simulink model "A_Identification_CSTR_open"  (R2024b)
settings: Solver=ode15s  StartTime=0.0  StopTime=100  RelTol=1e-3
settings Model: Creator=User  LastModifiedBy=HP
settings SolverCC: AlgebraicLoopSolver=TrustRegion
settings DebuggingCC: UnconnectedInputMsg=warning  UnconnectedOutputMsg=warning  UnconnectedLineMsg=warning
settings ModelReferenceCC: EnableRefExpFcnMdlSchedulingChecks=on
settings SFSimCC: CustomCodeUndefinedFunction=UseInterfaceOnly
settings RTWCC: GPUComputeCapability=3.5

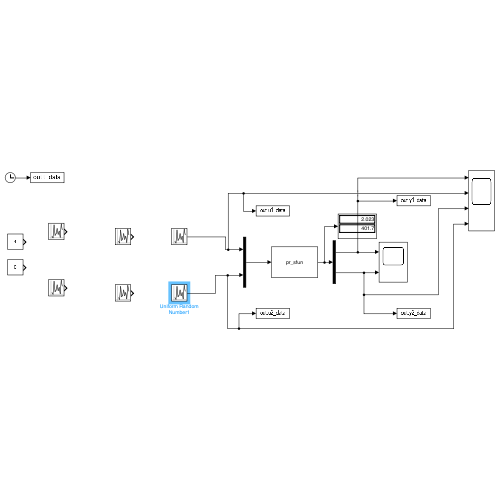
[thumbnail: Simulink's stored preview of the top-level diagram]
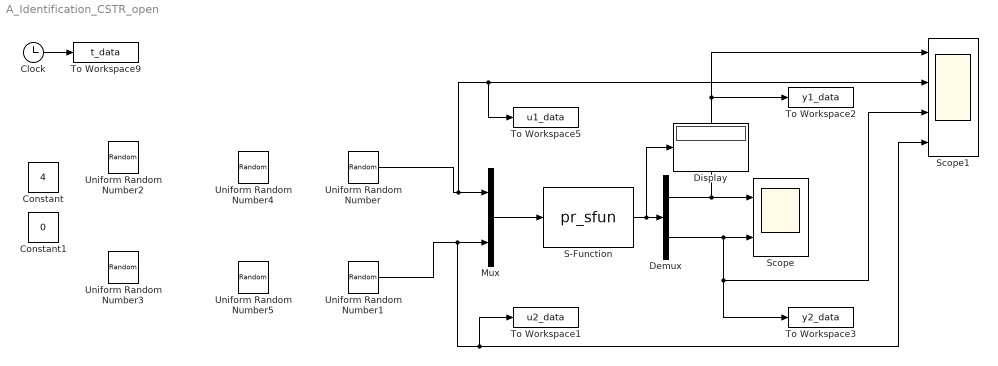
== system A_Identification_CSTR_open ==
  Clock : Clock
  Constant : Constant  Value=4
  Constant1 : Constant  Value=0
  Demux : Demux  Outputs=2
  Display : Display
  Mux : Mux  Inputs=2
  S-Function : S-Function  FunctionName=pr_sfun  SFunctionDeploymentMode=off  EnableBusSupport=off
  Scope : Scope  NumInputPorts=2
  Scope1 : Scope  NumInputPorts=4
  To Workspace1 : ToWorkspace  VariableName=u2_data  SampleTime=0.01
  To Workspace2 : ToWorkspace  VariableName=y1_data  SampleTime=0.01
  To Workspace3 : ToWorkspace  VariableName=y2_data  SampleTime=0.01
  To Workspace5 : ToWorkspace  VariableName=u1_data  SampleTime=0.01
  To Workspace9 : ToWorkspace  VariableName=t_data  SampleTime=0.01
  Uniform Random Number : UniformRandomNumber  Minimum=4-3.5  Maximum=4+1.7  SampleTime=0.1
  Uniform Random Number1 : UniformRandomNumber  Minimum=-0.01e4  Maximum=6e4  SampleTime=0.1
  Uniform Random Number2 : UniformRandomNumber  Minimum=4-3.5  Maximum=4+3.5  SampleTime=0.1
  Uniform Random Number3 : UniformRandomNumber  Minimum=-5e5  Maximum=5e5  SampleTime=0.1
  Uniform Random Number4 : UniformRandomNumber  Minimum=4-3.5  Maximum=4+3.5  SampleTime=0.1
  Uniform Random Number5 : UniformRandomNumber  Minimum=-5e3  Maximum=5e4  SampleTime=0.1
  wires:
  Demux/1 -> To Workspace2/1, Scope1/1, Scope/1
  Mux/1 -> S-Function/1
  S-Function/1 -> Display/1, Demux/1
  Demux/2 -> To Workspace3/1, Scope1/3, Scope/2
  Uniform Random Number/1 -> To Workspace5/1, Scope1/2, Mux/1
  Uniform Random Number1/1 -> To Workspace1/1, Scope1/4, Mux/2
  Clock/1 -> To Workspace9/1
